simulink model "RobustFormationControl_FractionalModel_under_Dis"  (R2023a)
settings: Solver=ode3  StartTime=0.0  StopTime=30  FixedStep=0.0001  RelTol=1e-3
InitFcn:
  | % close all;
  | % clear all;
  | % clc;
  | % System & Qaudrotor Parameters
  | %==============================
  | m = 0.486;                                         % Quadrotor Mass ( kg )
  | 
  | L = 0.25;                                         % Length of the arm ( m )
  | % L = 0.25;                                         % Length of the arm ( m )
  | 
  | Ixx = 4.856e-03; Iyy = 4.856e-03; Izz = 8.801e-03; % The moments of inertia around x,y and z axes respectively ( kg.m^2 )
  | % Ixx = 3.8278e-03; Iyy = 3.8278e-03; Izz = 7.6566e-03; % The moments of inertia around x,y and z axes respectively ( kg.m^2 )
  | 
  | Jr = 2.8385e-5;                                            % The inertia moment of rotor ( kg.m^2 )
  | % Jr = 0;
  | 
  | % Kx=5.5670e-4;
  | % Ky=5.5670e-4;
  | % Kz=6.3540e-4;
  | % kx=0.032;
  | % ky=0.032;
  | % kz=0.048;
  | Kfx = 5.5670e-4; Kfy = 5.5670e-4; Kfz = 6.3540e-4;% The Rotational drag cofficients ( N/rad/s )
  | 
  | % Ktx = 0.032; Kty = 0.032; Ktz = 0.048;               % The linear drag coefficients in x, y, z respectively ( N/m/s )
  | Ktx = 5.5670e-4; Kty =5.5670e-4; Ktz = 6.3540e-4;               % The linear drag coefficients in x, y, z respectively ( N/m/s )
  | 
  | b = 2.923e-05;                                      % The lift coefficient
  | % b = 2.9842e-05;                                      % The lift coefficient
  | 
  | d = 1.12e-06;                                       % The drag coefficient
  | % d = 3.2320e-07;                                       % The drag coefficient
  | 
  | g = 9.81;                                          % The acceleration due to gravity ( m/s^2 )
  | 
  | %-------- The Coefficients of Non-linear Equations of Quadrotor ( Page 11) -------
  | %--------------------------------------------------------------------------------
  | % Rotational Equations
  | %=====================
  | % Coefficients in ( eq1 ) >>..
  | a1 = (Iyy - Izz)/Ixx;
  | b1 = - Jr/Ixx;
  | c1 = - Kfx/Ixx;
  | d1 = L/Ixx;
  | 
  | % Coefficients in ( eq2 ) >>..
  | a2 = (Izz - Ixx)/Iyy;
  | b2 = Jr/Iyy;
  | c2 = - Kfy/Iyy;
  | d2 = L/Iyy;
  | 
  | % Coefficients in ( eq3 ) >>..
  | a3 = (Ixx - Iyy)/Izz;
  | b3 = - Kfz/Izz;
  | c3 = 1/Izz;
  | % c3 = d/Izz;
  | 
  | % Translational Equations
  | %========================
  | % Coefficients in ( eq4 ) >>..
  | a4 = - Ktx/m;
  | % a4 =0;
  | % b4 = L/m;
  | b4 = 1/m;
  | 
  | % Coefficients in ( eq5 ) >>..
  | a5 = - Kty/m;
  | b5 = 1/m;
  | % b5 = L/m;
  | 
  | % Coefficients in ( eq6 ) >>..
  | a6 = - Ktz/m;
  | % a6 = 0;
  | b6 = 1/m;
  | % b6 = L/m;
  | %=================
  | %=================
  | % Sliding Surfaces Parameters of Integer  Model - Rotational System >>...
  | % 10, 1
  | % 10, 0.1
  | k1 = 10; k2 = 0.01; % for S2 ( Roll Angle Sliding Surface  Param.) (200 , 0.5)
  | k3 = 10; k4 = 0.01; % for S4 ( Pitch Angle Sliding Surface  Param.)
  | k5 = 10; k6 = 0.01; % for S6 ( Yaw Angle Sliding Surface  Param.)
  | %--------------
  | 
  | % Sliding Modse Controller Parameters of Integer Model>>...
  | % 0.1 ; 20
  | % 100; 0.05
  | qPhi = 10; kPhi =150;  % for U2 (100,1)
  | qTheta = 10; kTheta = 150;  % for U3
  | qPsi = 10; kPsi = 150;  % for U4
  | %-----------------
  | %==========================================================================
  | %==========================================================================
  | % Sliding Surfaces Parameters of Fractional Model >>...
  | 
  | % S2, S4 and S6 have the same parameters of Sliding Surfaces with Integer Model
  | %--------------
  | % n = 0.1, nn = 0.1
  | % n = 0.5, nn = 10;
  | % n = 0.25, nn = 15;
  | 
  | % n = 0.3;
  | % nn = 21.3;
  | % (0.5, 50)
  | n = 0.01;
  | nn = 3;
  | % for S8 ( x Position Sliding Surfece  Param.) (500, 1)
  | % 10, 0.1
  | q7 = 1*nn; q8 = 1*n; q9 = 1*n; q10 = 1*n;
  | % for S10 ( y Position Sliding Surfece  Param.) (500, 1)
  | q11 = 1*nn; q12 = 1*n; q13 = 1*n; q14 = 1*n;
  | % for S12 ( z Position Sliding Surfece  Param.) (500, 1)
  | q15 = 1*nn; q16 = 1*n; q17 = 1*n; q18 = 1*n;
  | %-------------------------------------------------------------------------
  | % Sliding Mode Controller Parameters of Fractional Model>>...
  | % 0.1, 10
  | % 1, 15
  | % ( 10, 20)
  | gX = 1; sX = 200; % for Ux (10,100)
  | gY = 1; sY = 200; % for Uy (10,100)
  | gZ = 1; sZ = 200; % for U1 (10,100)
  | %-------------------------------------------------------------------------
  | %-------------------------------------------------------------------------
  | %-------------------------------------------------------------------------
  | %-------------------------------------------------------------------------
  | %-------------------------------------------------------------------------
  | %-------------------------------------------------------------------------
  | % Control Design Parameters for the followers:
  | %==============================================
  | % % Parameters for the fractional order NTFSMC:
  | % Sliding Surface " Sx, Sy, and Sz ":
  | %------------------------
  | cx = 50*[4 4 4];
  | cxx = 0.01*[0.01 0.01 0.01];
  | 
  | cx1 = cx(1);
  | cy1 = cx(2);
  | cz1 = cx(3);
  | 
  | cx2 = cxx(1);
  | cy2 = cxx(2);
  | cz2 = cxx(3);
  | 
  | alpha1 = [0.7 0.7 0.7];
  | alpha2 = [0.01 0.01 0.01];
  | 
  | gammaX = [4 4 4];
  | gx  = gammaX(1);
  | gy = gammaX(2);
  | gz = gammaX(3);
  | 
  | p = 10;
  | q = 10;
  | 
  | % Sliding Surface " S_Phi , S_Theta, and  S_Psi":
  | %------------------------
  | cP = 50*[4 4 4];
  | cPP = 0.10*[0.01 0.01 0.01 0.01];
  | 
  | cPhi1 = cP(1);
  | cTheta1 = cP(2);
  | cPsi1 = cP(3);
  | 
  | cPhi2 = cPP(1);
  | cTheta2 = cPP(2);
  | cPsi2 = cPP(3);
  | gammaP = [4 4 4];
  | 
  | %=========================
  | %=========================
  | SigmaX = 1*[0.01 0.01 0.01];
  | SigmaXX = 0.1*[1 1 1];
  | 
  | Sigma1X = SigmaX(1);
  | Sigma1Y = SigmaX(2);
  | Sigma1Z = SigmaX(3);
  | %-----
  | Sigma2X = SigmaXX(1);
  | Sigma2Y = SigmaXX(2);
  | Sigma2Z = SigmaXX(3);
  | 
  | 
  | SigmaP = 0.01*[0.01 0.01 0.01];
  | SigmaPP =100*[1 1 1];
  | 
  | Sigma1Phi   = SigmaP(1);
  | Sigma1Theta = SigmaP(2);
  | Sigma1Psi   = SigmaP(3);
  | %----
  | Sigma2Phi   = SigmaPP(1);
  | Sigma2Theta = SigmaPP(2);
  | Sigma2Psi   = SigmaPP(3);
  | 
  | q0 = 0.01;
  | q1 = 0.01;
  | q2 = 0.01;
  | w = 0;
  | %=========================================
  | %=========================================
  | %=========================================
  | %=========================================
  | %=========================================
  | %=========================================
  | %=========================================
  | %=========================================
  | % The value of Beta ( The fractional order of the FOSMCs)
  | Beta = 0.2;
  | % The value of Disturbance:
  | Dis = 1;
  | dis = 0;
libraries: fod x135, eeStairGenerator x5
(part 1 of 10)
settings Model: Creator=jofan  LastModifiedBy=jofan
settings DataIOCC: ReturnWorkspaceOutputs=off

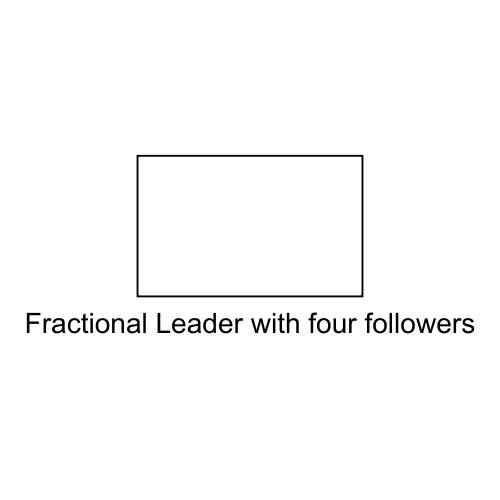
[thumbnail: Simulink's stored preview of the top-level diagram]
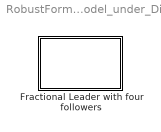
== system RobustFormationControl_FractionalModel_under_Dis ==
  Fractional Leader with four followers : Subsystem

== system RobustFormationControl_FractionalModel_under_Dis/Fractional Leader with four followers ==
  Follower 1 System : Subsystem
  Follower 2 System : Subsystem
  Follower 3 System : Subsystem
  Follower 4 System : Subsystem
  Fractional Model of the Leader : Subsystem
  Mux{,1..3} (4 alike) : Mux  Inputs=3
  dX : Constant  Value=-2
  dX1 : Constant  Value=-2
  dX2 : Constant  Value=-4
  dX3 : Constant  Value=-4
  dY : Constant  Value=2
  dY1 : Constant  Value=-2
  dY2 : Constant  Value=4
  dY3 : Constant  Value=-4
  dZ{,1..3} (4 alike) : Constant  Value=0
  wires:
  dY/1 -> Mux/2
  dZ/1 -> Mux/3
  dX/1 -> Mux/1
  dY1/1 -> Mux1/2
  dZ1/1 -> Mux1/3
  dX1/1 -> Mux1/1
  dX2/1 -> Mux2/1
  dZ2/1 -> Mux2/3
  dY2/1 -> Mux2/2
  dY3/1 -> Mux3/2
  dZ3/1 -> Mux3/3
  dX3/1 -> Mux3/1
  Mux/1 -> [dXYZ]
  Mux1/1 -> [dXYZ1]
  Mux2/1 -> [dXYZ2]
  Mux3/1 -> [dXYZ3]
  Fractional Model of the Leader/1(xLeader) -> [xyzL]
  [xyzL] -> Follower 1 System/1(xLeader)
  [xyzL] -> Follower 2 System/1(xLeader)
  [xyzL] -> Follower 4 System/1(xLeader)
  [xyzL] -> Follower 3 System/1(xLeader)
  [dXYZ] -> Follower 1 System/2(dXYZ)
  [dXYZ2] -> Follower 3 System/2(dXYZ)
  [dXYZ1] -> Follower 2 System/2(dXYZ)
  [dXYZ3] -> Follower 4 System/2(dXYZ)

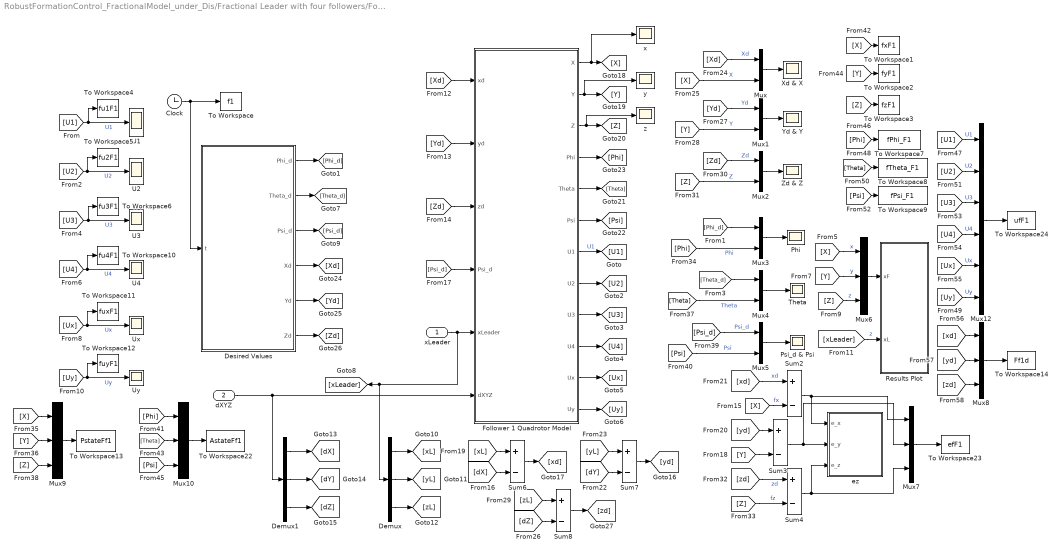
== system RobustFormationControl_FractionalModel_under_Dis/Fractional Leader with four followers/Follower 1 System ==
  xLeader : Inport
  dXYZ : Inport  Port=2
  " Phi " : Scope
  Clock : Clock
  Demux : Demux  Outputs=3
  Demux1 : Demux  Outputs=3
  Desired Values : Subsystem
  Follower 1 Quadrotor Model : Subsystem
  Mux{,1..5} (6 alike) : Mux  Inputs=2
  Mux{6..10} (5 alike) : Mux  Inputs=3
  Mux12 : Mux  Inputs=6
  Psi_d & Psi : Scope
  Results Plot : Subsystem
  Sum{2..4,6..8} (6 alike) : Sum  Inputs=+-
  "Theta " : Scope
  To Workspace : ToWorkspace  VariableName=f1  SampleTime=0.03
  To Workspace1 : ToWorkspace  VariableName=fxF1  SampleTime=0.03
  To Workspace10 : ToWorkspace  VariableName=fu4F1  SampleTime=0.03
  To Workspace11 : ToWorkspace  VariableName=fuxF1  SampleTime=0.03
  To Workspace12 : ToWorkspace  VariableName=fuyF1  SampleTime=0.03
  To Workspace13 : ToWorkspace  VariableName=PstateFf1  SampleTime=-1
  To Workspace14 : ToWorkspace  VariableName=Ff1d  SampleTime=-1
  To Workspace2 : ToWorkspace  VariableName=fyF1  SampleTime=0.03
  To Workspace22 : ToWorkspace  VariableName=AstateFf1  SampleTime=-1
  To Workspace23 : ToWorkspace  VariableName=efF1  SampleTime=-1
  To Workspace24 : ToWorkspace  VariableName=ufF1  SampleTime=-1
  To Workspace3 : ToWorkspace  VariableName=fzF1  SampleTime=0.03
  To Workspace4 : ToWorkspace  VariableName=fu1F1  SampleTime=0.03
  To Workspace5 : ToWorkspace  VariableName=fu2F1  SampleTime=0.03
  To Workspace6 : ToWorkspace  VariableName=fu3F1  SampleTime=0.03
  To Workspace7 : ToWorkspace  VariableName=fPhi_F1  SampleTime=0.03
  To Workspace8 : ToWorkspace  VariableName=fTheta_F1  SampleTime=0.03
  To Workspace9 : ToWorkspace  VariableName=fPsi_F1  SampleTime=0.03
  "U1 " : Scope
  U2 : Scope
  "U3 " : Scope
  "U4 " : Scope
  Ux : Scope
  Uy : Scope
  "Xd & X " : Scope
  Yd & Y : Scope
  "Zd & Z " : Scope
  ez : Subsystem
  x : Scope
  y : Scope
  z : Scope
  wires:
  Mux4/1 -> "Theta "/1
  [U2] -> To Workspace5/1, U2/1  "U2"
  [Yd] -> Mux1/1  "Yd"
  Follower 1 Quadrotor Model/10(U4) -> [U4]
  [Zd] -> Follower 1 Quadrotor Model/3(zd)
  [U4] -> To Workspace10/1, "U4 "/1  "U4"
  [Psi] -> To Workspace9/1
  [Z] -> Mux2/2  "Z"
  Follower 1 Quadrotor Model/2(Y) -> y/1, [Y]
  Clock/1 -> To Workspace/1, Desired Values/1(t)
  Follower 1 Quadrotor Model/7(U1) -> [U1]  "U1"
  Desired Values/2(Theta_d) -> [Theta_d]
  Mux2/1 -> "Zd & Z "/1
  [Theta] -> To Workspace8/1
  [Xd] -> Mux/1  "Xd"
  Follower 1 Quadrotor Model/12(Uy) -> [Uy]
  [Y] -> To Workspace2/1
  Follower 1 Quadrotor Model/11(Ux) -> [Ux]
  [X] -> To Workspace1/1
  [Yd] -> Follower 1 Quadrotor Model/2(yd)
  Mux/1 -> "Xd & X "/1
  Follower 1 Quadrotor Model/1(X) -> x/1, [X]
  Mux3/1 -> " Phi "/1
  Follower 1 Quadrotor Model/5(Theta) -> [Theta]
  Mux5/1 -> Psi_d & Psi/1
  [X] -> Mux/2  "X"
  Follower 1 Quadrotor Model/9(U3) -> [U3]
  [Theta] -> Mux4/2  "Theta"
  [Y] -> Mux1/2  "Y"
  [Uy] -> To Workspace12/1, Uy/1  "Uy"
  Desired Values/3(Psi_d) -> [Psi_d]
  Follower 1 Quadrotor Model/3(Z) -> z/1, [Z]
  [U1] -> To Workspace4/1, "U1 "/1  "U1"
  [Ux] -> To Workspace11/1, Ux/1  "Ux"
  Desired Values/6(Zd) -> [Zd]
  [Phi] -> Mux3/2  "Phi"
  Mux1/1 -> Yd & Y/1
  [Xd] -> Follower 1 Quadrotor Model/1(xd)
  [Psi] -> Mux5/2  "Psi"
  [Z] -> To Workspace3/1
  Follower 1 Quadrotor Model/8(U2) -> [U2]
  [Theta_d] -> Mux4/1
  [Psi_d] -> Mux5/1  "Psi_d"
  [Zd] -> Mux2/1  "Zd"
  [U3] -> To Workspace6/1, "U3 "/1  "U3"
  Desired Values/5(Yd) -> [Yd]
  [Psi_d] -> Follower 1 Quadrotor Model/4(Psi_d)
  Follower 1 Quadrotor Model/6(Psi) -> [Psi]
  Follower 1 Quadrotor Model/4(Phi) -> [Phi]
  Desired Values/4(Xd) -> [Xd]
  [Phi_d] -> Mux3/1
  Desired Values/1(Phi_d) -> [Phi_d]
  [Phi] -> To Workspace7/1
  xLeader/1 -> Demux/1, [xLeader], Follower 1 Quadrotor Model/5(xLeader)
  [Z] -> Mux6/3  "z"
  [X] -> Mux6/1  "x"
  [xLeader] -> Results Plot/2(xL)  "z"
  Mux6/1 -> Results Plot/1(xF)
  [Y] -> Mux6/2  "y"
  dXYZ/1 -> Demux1/1, Follower 1 Quadrotor Model/6(dXYZ)
  Demux/1 -> [xL]
  Demux/3 -> [zL]
  Demux/2 -> [yL]
  Demux1/3 -> [dZ]
  Demux1/2 -> [dY]
  Demux1/1 -> [dX]
  [xL] -> Sum6/1
  [dX] -> Sum6/2
  [dY] -> Sum7/2
  [yL] -> Sum7/1
  [dZ] -> Sum8/2
  [zL] -> Sum8/1
  Sum7/1 -> [yd]
  Sum6/1 -> [xd]
  Sum8/1 -> [zd]
  [yd] -> Mux8/2
  [zd] -> Sum4/1  "zd"
  [Z] -> Mux9/3
  [Uy] -> Mux12/6  "Uy"
  [Z] -> Sum4/2  "fz"
  [X] -> Mux9/1
  [U2] -> Mux12/2  "U2"
  [Ux] -> Mux12/5  "Ux"
  [U1] -> Mux12/1  "U1"
  [Y] -> Mux9/2
  Sum3/1 -> Mux7/2, ez/2(e_y)
  [Y] -> Sum3/2
  Sum2/1 -> Mux7/1, ez/1(e_x)
  Sum4/1 -> Mux7/3, ez/3(e_z)
  [yd] -> Sum3/1
  Mux12/1 -> To Workspace24/1
  [Theta] -> Mux10/2
  [Psi] -> Mux10/3
  Mux7/1 -> To Workspace23/1
  [zd] -> Mux8/3
  Mux8/1 -> To Workspace14/1
  [X] -> Sum2/2  "fx"
  Mux10/1 -> To Workspace22/1
  Mux9/1 -> To Workspace13/1
  [Phi] -> Mux10/1
  [U4] -> Mux12/4  "U4"
  [xd] -> Mux8/1
  [U3] -> Mux12/3  "U3"
  [xd] -> Sum2/1  "xd"

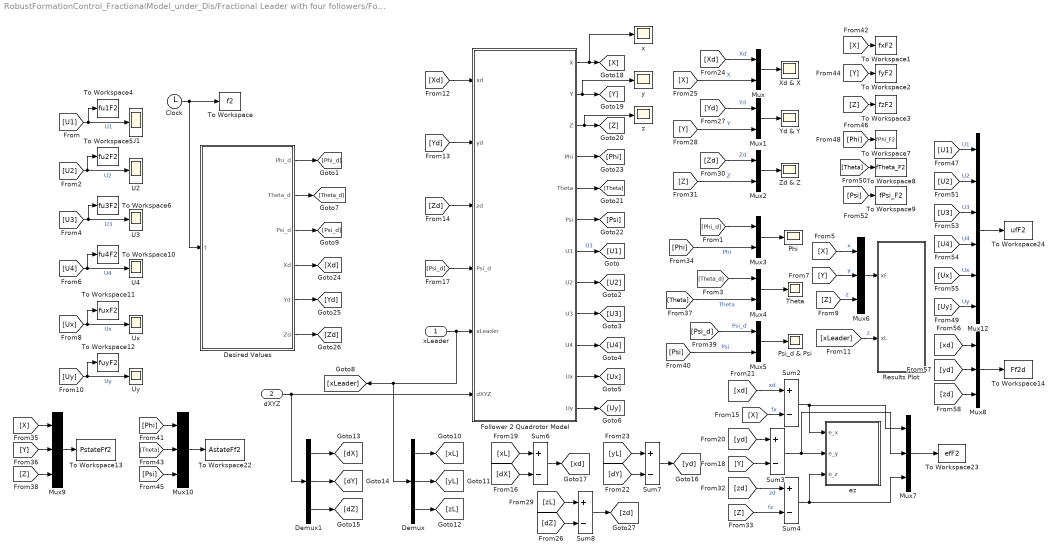
== system RobustFormationControl_FractionalModel_under_Dis/Fractional Leader with four followers/Follower 2 System ==
  xLeader : Inport
  dXYZ : Inport  Port=2
  " Phi " : Scope
  Clock : Clock
  Demux : Demux  Outputs=3
  Demux1 : Demux  Outputs=3
  Desired Values : Subsystem
  Follower 2 Quadrotor Model : Subsystem
  Mux{,1..5} (6 alike) : Mux  Inputs=2
  Mux{6..10} (5 alike) : Mux  Inputs=3
  Mux12 : Mux  Inputs=6
  Psi_d & Psi : Scope
  Results Plot : Subsystem
  Sum{2..4,6..8} (6 alike) : Sum  Inputs=+-
  "Theta " : Scope
  To Workspace : ToWorkspace  VariableName=f2  SampleTime=0.03
  To Workspace1 : ToWorkspace  VariableName=fxF2  SampleTime=0.03
  To Workspace10 : ToWorkspace  VariableName=fu4F2  SampleTime=0.03
  To Workspace11 : ToWorkspace  VariableName=fuxF2  SampleTime=0.03
  To Workspace12 : ToWorkspace  VariableName=fuyF2  SampleTime=0.03
  To Workspace13 : ToWorkspace  VariableName=PstateFf2  SampleTime=-1
  To Workspace14 : ToWorkspace  VariableName=Ff2d  SampleTime=-1
  To Workspace2 : ToWorkspace  VariableName=fyF2  SampleTime=0.03
  To Workspace22 : ToWorkspace  VariableName=AstateFf2  SampleTime=-1
  To Workspace23 : ToWorkspace  VariableName=efF2  SampleTime=-1
  To Workspace24 : ToWorkspace  VariableName=ufF2  SampleTime=-1
  To Workspace3 : ToWorkspace  VariableName=fzF2  SampleTime=0.03
  To Workspace4 : ToWorkspace  VariableName=fu1F2  SampleTime=0.03
  To Workspace5 : ToWorkspace  VariableName=fu2F2  SampleTime=0.03
  To Workspace6 : ToWorkspace  VariableName=fu3F2  SampleTime=0.03
  To Workspace7 : ToWorkspace  VariableName=fPhi_F2  SampleTime=0.03
  To Workspace8 : ToWorkspace  VariableName=fTheta_F2  SampleTime=0.03
  To Workspace9 : ToWorkspace  VariableName=fPsi_F2  SampleTime=0.03
  "U1 " : Scope
  U2 : Scope
  "U3 " : Scope
  "U4 " : Scope
  Ux : Scope
  Uy : Scope
  "Xd & X " : Scope
  Yd & Y : Scope
  "Zd & Z " : Scope
  ez : Subsystem
  x : Scope
  y : Scope
  z : Scope
  wires:
  Mux4/1 -> "Theta "/1
  [U2] -> To Workspace5/1, U2/1  "U2"
  [Yd] -> Mux1/1  "Yd"
  Follower 2 Quadrotor Model/10(U4) -> [U4]
  [Zd] -> Follower 2 Quadrotor Model/3(zd)
  [U4] -> To Workspace10/1, "U4 "/1  "U4"
  [Psi] -> To Workspace9/1
  [Z] -> Mux2/2  "Z"
  Follower 2 Quadrotor Model/2(Y) -> y/1, [Y]
  Clock/1 -> To Workspace/1, Desired Values/1(t)
  Follower 2 Quadrotor Model/7(U1) -> [U1]  "U1"
  Desired Values/2(Theta_d) -> [Theta_d]
  Mux2/1 -> "Zd & Z "/1
  [Theta] -> To Workspace8/1
  [Xd] -> Mux/1  "Xd"
  Follower 2 Quadrotor Model/12(Uy) -> [Uy]
  [Y] -> To Workspace2/1
  Follower 2 Quadrotor Model/11(Ux) -> [Ux]
  [X] -> To Workspace1/1
  [Yd] -> Follower 2 Quadrotor Model/2(yd)
  Mux/1 -> "Xd & X "/1
  Follower 2 Quadrotor Model/1(X) -> x/1, [X]
  Mux3/1 -> " Phi "/1
  Follower 2 Quadrotor Model/5(Theta) -> [Theta]
  Mux5/1 -> Psi_d & Psi/1
  [X] -> Mux/2  "X"
  Follower 2 Quadrotor Model/9(U3) -> [U3]
  [Theta] -> Mux4/2  "Theta"
  [Y] -> Mux1/2  "Y"
  [Uy] -> To Workspace12/1, Uy/1  "Uy"
  Desired Values/3(Psi_d) -> [Psi_d]
  Follower 2 Quadrotor Model/3(Z) -> z/1, [Z]
  [U1] -> To Workspace4/1, "U1 "/1  "U1"
  [Ux] -> To Workspace11/1, Ux/1  "Ux"
  Desired Values/6(Zd) -> [Zd]
  [Phi] -> Mux3/2  "Phi"
  Mux1/1 -> Yd & Y/1
  [Xd] -> Follower 2 Quadrotor Model/1(xd)
  [Psi] -> Mux5/2  "Psi"
  [Z] -> To Workspace3/1
  Follower 2 Quadrotor Model/8(U2) -> [U2]
  [Theta_d] -> Mux4/1
  [Psi_d] -> Mux5/1  "Psi_d"
  [Zd] -> Mux2/1  "Zd"
  [U3] -> To Workspace6/1, "U3 "/1  "U3"
  Desired Values/5(Yd) -> [Yd]
  [Psi_d] -> Follower 2 Quadrotor Model/4(Psi_d)
  Follower 2 Quadrotor Model/6(Psi) -> [Psi]
  Follower 2 Quadrotor Model/4(Phi) -> [Phi]
  Desired Values/4(Xd) -> [Xd]
  [Phi_d] -> Mux3/1
  Desired Values/1(Phi_d) -> [Phi_d]
  [Phi] -> To Workspace7/1
  [Z] -> Mux6/3  "z"
  [X] -> Mux6/1  "x"
  [xLeader] -> Results Plot/2(xL)  "z"
  Mux6/1 -> Results Plot/1(xF)
  [Y] -> Mux6/2  "y"
  Demux1/3 -> [dZ]
  Demux/2 -> [yL]
  Sum8/1 -> [zd]
  [dZ] -> Sum8/2
  [dX] -> Sum6/2
  dXYZ/1 -> Demux1/1, Follower 2 Quadrotor Model/6(dXYZ)
  [zL] -> Sum8/1
  Sum7/1 -> [yd]
  [yL] -> Sum7/1
  Demux/3 -> [zL]
  [dY] -> Sum7/2
  Demux1/1 -> [dX]
  Demux/1 -> [xL]
  Sum6/1 -> [xd]
  xLeader/1 -> [xLeader], Demux/1, Follower 2 Quadrotor Model/5(xLeader)
  Demux1/2 -> [dY]
  [xL] -> Sum6/1
  [Z] -> Mux9/3
  [zd] -> Sum4/1  "zd"
  [Phi] -> Mux10/1
  [U3] -> Mux12/3  "U3"
  [xd] -> Mux8/1
  Mux9/1 -> To Workspace13/1
  [Theta] -> Mux10/2
  Mux7/1 -> To Workspace23/1
  [X] -> Sum2/2  "fx"
  [Psi] -> Mux10/3
  Mux8/1 -> To Workspace14/1
  Sum2/1 -> Mux7/1, ez/1(e_x)
  [U4] -> Mux12/4  "U4"
  Sum4/1 -> Mux7/3, ez/3(e_z)
  Mux12/1 -> To Workspace24/1
  Sum3/1 -> Mux7/2, ez/2(e_y)
  [Y] -> Sum3/2
  Mux10/1 -> To Workspace22/1
  [U2] -> Mux12/2  "U2"
  [zd] -> Mux8/3
  [Y] -> Mux9/2
  [Ux] -> Mux12/5  "Ux"
  [yd] -> Mux8/2
  [X] -> Mux9/1
  [Uy] -> Mux12/6  "Uy"
  [yd] -> Sum3/1
  [U1] -> Mux12/1  "U1"
  [Z] -> Sum4/2  "fz"
  [xd] -> Sum2/1  "xd"

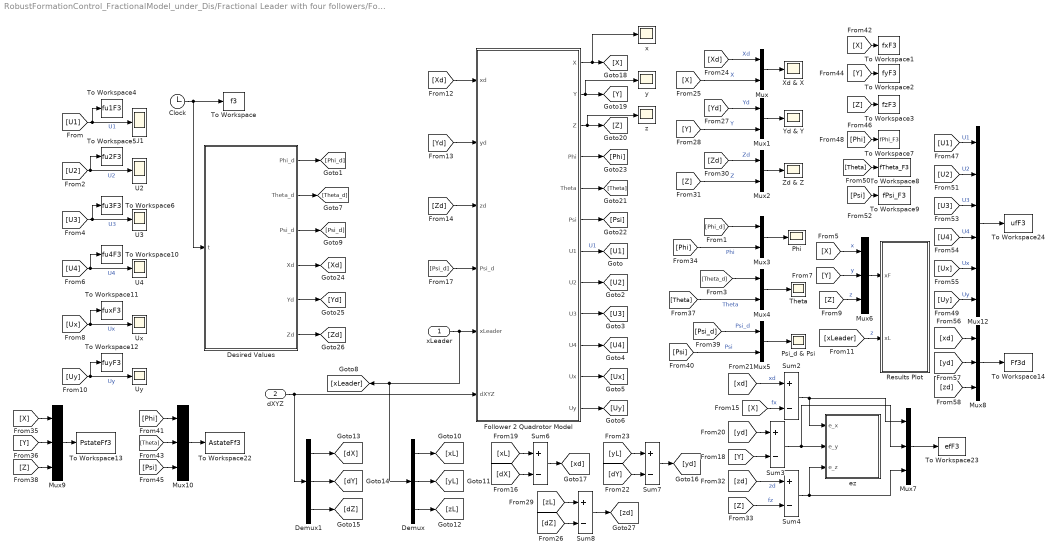
== system RobustFormationControl_FractionalModel_under_Dis/Fractional Leader with four followers/Follower 3 System ==
  xLeader : Inport
  dXYZ : Inport  Port=2
  " Phi " : Scope
  Clock : Clock
  Demux : Demux  Outputs=3
  Demux1 : Demux  Outputs=3
  Desired Values : Subsystem
  Follower 2 Quadrotor Model : Subsystem
  Mux{,1..5} (6 alike) : Mux  Inputs=2
  Mux{6..10} (5 alike) : Mux  Inputs=3
  Mux12 : Mux  Inputs=6
  Psi_d & Psi : Scope
  Results Plot : Subsystem
  Sum{2..4,6..8} (6 alike) : Sum  Inputs=+-
  "Theta " : Scope
  To Workspace : ToWorkspace  VariableName=f3  SampleTime=0.03
  To Workspace1 : ToWorkspace  VariableName=fxF3  SampleTime=0.03
  To Workspace10 : ToWorkspace  VariableName=fu4F3  SampleTime=0.03
  To Workspace11 : ToWorkspace  VariableName=fuxF3  SampleTime=0.03
  To Workspace12 : ToWorkspace  VariableName=fuyF3  SampleTime=0.03
  To Workspace13 : ToWorkspace  VariableName=PstateFf3  SampleTime=-1
  To Workspace14 : ToWorkspace  VariableName=Ff3d  SampleTime=-1
  To Workspace2 : ToWorkspace  VariableName=fyF3  SampleTime=0.03
  To Workspace22 : ToWorkspace  VariableName=AstateFf3  SampleTime=-1
  To Workspace23 : ToWorkspace  VariableName=efF3  SampleTime=-1
  To Workspace24 : ToWorkspace  VariableName=ufF3  SampleTime=-1
  To Workspace3 : ToWorkspace  VariableName=fzF3  SampleTime=0.03
  To Workspace4 : ToWorkspace  VariableName=fu1F3  SampleTime=0.03
  To Workspace5 : ToWorkspace  VariableName=fu2F3  SampleTime=0.03
  To Workspace6 : ToWorkspace  VariableName=fu3F3  SampleTime=0.03
  To Workspace7 : ToWorkspace  VariableName=fPhi_F3  SampleTime=0.03
  To Workspace8 : ToWorkspace  VariableName=fTheta_F3  SampleTime=0.03
  To Workspace9 : ToWorkspace  VariableName=fPsi_F3  SampleTime=0.03
  "U1 " : Scope
  U2 : Scope
  "U3 " : Scope
  "U4 " : Scope
  Ux : Scope
  Uy : Scope
  "Xd & X " : Scope
  Yd & Y : Scope
  "Zd & Z " : Scope
  ez : Subsystem
  x : Scope
  y : Scope
  z : Scope
  wires:
  [Y] -> Mux6/2  "y"
  Mux6/1 -> Results Plot/1(xF)
  [xLeader] -> Results Plot/2(xL)  "z"
  [X] -> Mux6/1  "x"
  [Z] -> Mux6/3  "z"
  xLeader/1 -> Follower 2 Quadrotor Model/5(xLeader), Demux/1, [xLeader]
  [Phi] -> To Workspace7/1
  Desired Values/1(Phi_d) -> [Phi_d]
  [Phi_d] -> Mux3/1
  Desired Values/4(Xd) -> [Xd]
  Follower 2 Quadrotor Model/4(Phi) -> [Phi]
  Follower 2 Quadrotor Model/6(Psi) -> [Psi]
  [Psi_d] -> Follower 2 Quadrotor Model/4(Psi_d)
  Desired Values/5(Yd) -> [Yd]
  [U3] -> "U3 "/1, To Workspace6/1  "U3"
  [Zd] -> Mux2/1  "Zd"
  [Psi_d] -> Mux5/1  "Psi_d"
  [Theta_d] -> Mux4/1
  Follower 2 Quadrotor Model/8(U2) -> [U2]
  [Z] -> To Workspace3/1
  [Psi] -> Mux5/2  "Psi"
  [Xd] -> Follower 2 Quadrotor Model/1(xd)
  Mux1/1 -> Yd & Y/1
  [Phi] -> Mux3/2  "Phi"
  Desired Values/6(Zd) -> [Zd]
  [Ux] -> Ux/1, To Workspace11/1  "Ux"
  [U1] -> "U1 "/1, To Workspace4/1  "U1"
  Follower 2 Quadrotor Model/3(Z) -> [Z], z/1
  Desired Values/3(Psi_d) -> [Psi_d]
  [Uy] -> Uy/1, To Workspace12/1  "Uy"
  [Y] -> Mux1/2  "Y"
  [Theta] -> Mux4/2  "Theta"
  Follower 2 Quadrotor Model/9(U3) -> [U3]
  [X] -> Mux/2  "X"
  Mux5/1 -> Psi_d & Psi/1
  Follower 2 Quadrotor Model/5(Theta) -> [Theta]
  Mux3/1 -> " Phi "/1
  Follower 2 Quadrotor Model/1(X) -> [X], x/1
  Mux/1 -> "Xd & X "/1
  [Yd] -> Follower 2 Quadrotor Model/2(yd)
  [X] -> To Workspace1/1
  Follower 2 Quadrotor Model/11(Ux) -> [Ux]
  [Y] -> To Workspace2/1
  Follower 2 Quadrotor Model/12(Uy) -> [Uy]
  [Xd] -> Mux/1  "Xd"
  [Theta] -> To Workspace8/1
  Mux2/1 -> "Zd & Z "/1
  Desired Values/2(Theta_d) -> [Theta_d]
  Follower 2 Quadrotor Model/7(U1) -> [U1]  "U1"
  Clock/1 -> Desired Values/1(t), To Workspace/1
  Follower 2 Quadrotor Model/2(Y) -> [Y], y/1
  [Z] -> Mux2/2  "Z"
  [Psi] -> To Workspace9/1
  [U4] -> "U4 "/1, To Workspace10/1  "U4"
  [Zd] -> Follower 2 Quadrotor Model/3(zd)
  Follower 2 Quadrotor Model/10(U4) -> [U4]
  [Yd] -> Mux1/1  "Yd"
  [U2] -> U2/1, To Workspace5/1  "U2"
  Mux4/1 -> "Theta "/1
  Demux1/3 -> [dZ]
  Demux/2 -> [yL]
  Sum8/1 -> [zd]
  [dZ] -> Sum8/2
  [dX] -> Sum6/2
  dXYZ/1 -> Demux1/1, Follower 2 Quadrotor Model/6(dXYZ)
  [zL] -> Sum8/1
  Sum7/1 -> [yd]
  [yL] -> Sum7/1
  Demux/3 -> [zL]
  [dY] -> Sum7/2
  Demux1/1 -> [dX]
  Demux/1 -> [xL]
  Sum6/1 -> [xd]
  Demux1/2 -> [dY]
  [xL] -> Sum6/1
  [Z] -> Mux9/3
  [zd] -> Sum4/1  "zd"
  [Phi] -> Mux10/1
  [U3] -> Mux12/3  "U3"
  [xd] -> Mux8/1
  Mux9/1 -> To Workspace13/1
  [Theta] -> Mux10/2
  Mux7/1 -> To Workspace23/1
  [X] -> Sum2/2  "fx"
  [Psi] -> Mux10/3
  Mux8/1 -> To Workspace14/1
  Sum2/1 -> Mux7/1, ez/1(e_x)
  [U4] -> Mux12/4  "U4"
  Sum4/1 -> Mux7/3, ez/3(e_z)
  Mux12/1 -> To Workspace24/1
  Sum3/1 -> Mux7/2, ez/2(e_y)
  [Y] -> Sum3/2
  Mux10/1 -> To Workspace22/1
  [U2] -> Mux12/2  "U2"
  [zd] -> Mux8/3
  [Y] -> Mux9/2
  [Ux] -> Mux12/5  "Ux"
  [yd] -> Mux8/2
  [X] -> Mux9/1
  [Uy] -> Mux12/6  "Uy"
  [yd] -> Sum3/1
  [U1] -> Mux12/1  "U1"
  [Z] -> Sum4/2  "fz"
  [xd] -> Sum2/1  "xd"

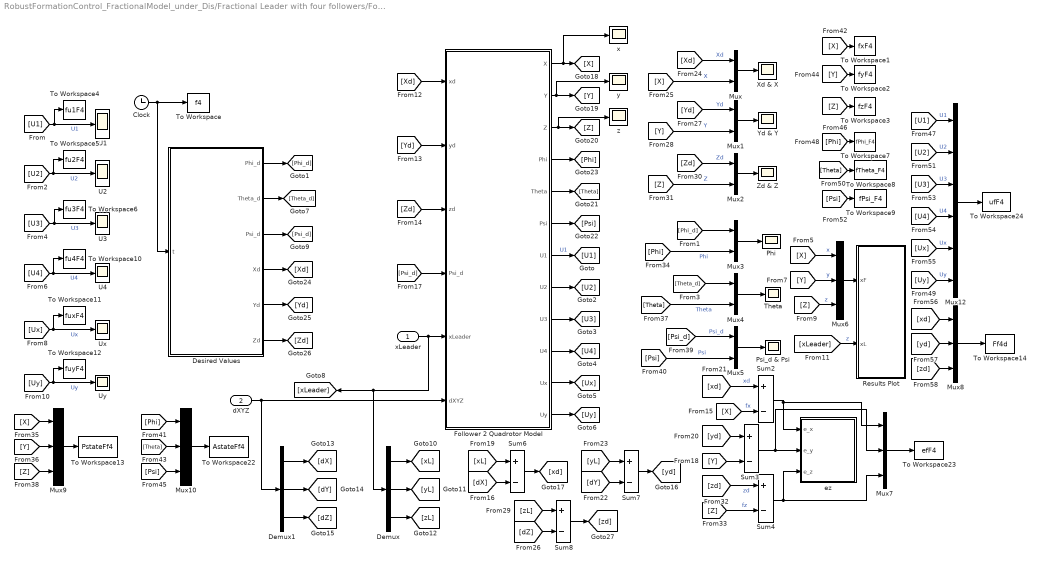
== system RobustFormationControl_FractionalModel_under_Dis/Fractional Leader with four followers/Follower 4 System ==
  xLeader : Inport
  dXYZ : Inport  Port=2
  " Phi " : Scope
  Clock : Clock
  Demux : Demux  Outputs=3
  Demux1 : Demux  Outputs=3
  Desired Values : Subsystem
  Follower 2 Quadrotor Model : Subsystem
  Mux{,1..5} (6 alike) : Mux  Inputs=2
  Mux{6..10} (5 alike) : Mux  Inputs=3
  Mux12 : Mux  Inputs=6
  Psi_d & Psi : Scope
  Results Plot : Subsystem
  Sum{2..4,6..8} (6 alike) : Sum  Inputs=+-
  "Theta " : Scope
  To Workspace : ToWorkspace  VariableName=f4  SampleTime=0.03
  To Workspace1 : ToWorkspace  VariableName=fxF4  SampleTime=0.03
  To Workspace10 : ToWorkspace  VariableName=fu4F4  SampleTime=0.03
  To Workspace11 : ToWorkspace  VariableName=fuxF4  SampleTime=0.03
  To Workspace12 : ToWorkspace  VariableName=fuyF4  SampleTime=0.03
  To Workspace13 : ToWorkspace  VariableName=PstateFf4  SampleTime=-1
  To Workspace14 : ToWorkspace  VariableName=Ff4d  SampleTime=-1
  To Workspace2 : ToWorkspace  VariableName=fyF4  SampleTime=0.03
  To Workspace22 : ToWorkspace  VariableName=AstateFf4  SampleTime=-1
  To Workspace23 : ToWorkspace  VariableName=efF4  SampleTime=-1
  To Workspace24 : ToWorkspace  VariableName=ufF4  SampleTime=-1
  To Workspace3 : ToWorkspace  VariableName=fzF4  SampleTime=0.03
  To Workspace4 : ToWorkspace  VariableName=fu1F4  SampleTime=0.03
  To Workspace5 : ToWorkspace  VariableName=fu2F4  SampleTime=0.03
  To Workspace6 : ToWorkspace  VariableName=fu3F4  SampleTime=0.03
  To Workspace7 : ToWorkspace  VariableName=fPhi_F4  SampleTime=0.03
  To Workspace8 : ToWorkspace  VariableName=fTheta_F4  SampleTime=0.03
  To Workspace9 : ToWorkspace  VariableName=fPsi_F4  SampleTime=0.03
  "U1 " : Scope
  U2 : Scope
  "U3 " : Scope
  "U4 " : Scope
  Ux : Scope
  Uy : Scope
  "Xd & X " : Scope
  Yd & Y : Scope
  "Zd & Z " : Scope
  ez : Subsystem
  x : Scope
  y : Scope
  z : Scope
  wires:
  Mux4/1 -> "Theta "/1
  [U2] -> To Workspace5/1, U2/1  "U2"
  [Yd] -> Mux1/1  "Yd"
  Follower 2 Quadrotor Model/10(U4) -> [U4]
  [Zd] -> Follower 2 Quadrotor Model/3(zd)
  [U4] -> To Workspace10/1, "U4 "/1  "U4"
  [Psi] -> To Workspace9/1
  [Z] -> Mux2/2  "Z"
  Follower 2 Quadrotor Model/2(Y) -> y/1, [Y]
  Clock/1 -> To Workspace/1, Desired Values/1(t)
  Follower 2 Quadrotor Model/7(U1) -> [U1]  "U1"
  Desired Values/2(Theta_d) -> [Theta_d]
  Mux2/1 -> "Zd & Z "/1
  [Theta] -> To Workspace8/1
  [Xd] -> Mux/1  "Xd"
  Follower 2 Quadrotor Model/12(Uy) -> [Uy]
  [Y] -> To Workspace2/1
  Follower 2 Quadrotor Model/11(Ux) -> [Ux]
  [X] -> To Workspace1/1
  [Yd] -> Follower 2 Quadrotor Model/2(yd)
  Mux/1 -> "Xd & X "/1
  Follower 2 Quadrotor Model/1(X) -> x/1, [X]
  Mux3/1 -> " Phi "/1
  Follower 2 Quadrotor Model/5(Theta) -> [Theta]
  Mux5/1 -> Psi_d & Psi/1
  [X] -> Mux/2  "X"
  Follower 2 Quadrotor Model/9(U3) -> [U3]
  [Theta] -> Mux4/2  "Theta"
  [Y] -> Mux1/2  "Y"
  [Uy] -> To Workspace12/1, Uy/1  "Uy"
  Desired Values/3(Psi_d) -> [Psi_d]
  Follower 2 Quadrotor Model/3(Z) -> z/1, [Z]
  [U1] -> To Workspace4/1, "U1 "/1  "U1"
  [Ux] -> To Workspace11/1, Ux/1  "Ux"
  Desired Values/6(Zd) -> [Zd]
  [Phi] -> Mux3/2  "Phi"
  Mux1/1 -> Yd & Y/1
  [Xd] -> Follower 2 Quadrotor Model/1(xd)
  [Psi] -> Mux5/2  "Psi"
  [Z] -> To Workspace3/1
  Follower 2 Quadrotor Model/8(U2) -> [U2]
  [Theta_d] -> Mux4/1
  [Psi_d] -> Mux5/1  "Psi_d"
  [Zd] -> Mux2/1  "Zd"
  [U3] -> To Workspace6/1, "U3 "/1  "U3"
  Desired Values/5(Yd) -> [Yd]
  [Psi_d] -> Follower 2 Quadrotor Model/4(Psi_d)
  Follower 2 Quadrotor Model/6(Psi) -> [Psi]
  Follower 2 Quadrotor Model/4(Phi) -> [Phi]
  Desired Values/4(Xd) -> [Xd]
  [Phi_d] -> Mux3/1
  Desired Values/1(Phi_d) -> [Phi_d]
  [Phi] -> To Workspace7/1
  xLeader/1 -> Demux/1, [xLeader], Follower 2 Quadrotor Model/5(xLeader)
  [Z] -> Mux6/3  "z"
  [X] -> Mux6/1  "x"
  [xLeader] -> Results Plot/2(xL)  "z"
  Mux6/1 -> Results Plot/1(xF)
  [Y] -> Mux6/2  "y"
  Demux1/3 -> [dZ]
  Demux/2 -> [yL]
  Sum8/1 -> [zd]
  [dZ] -> Sum8/2
  [dX] -> Sum6/2
  dXYZ/1 -> Demux1/1, Follower 2 Quadrotor Model/6(dXYZ)
  [zL] -> Sum8/1
  Sum7/1 -> [yd]
  [yL] -> Sum7/1
  Demux/3 -> [zL]
  [dY] -> Sum7/2
  Demux1/1 -> [dX]
  Demux/1 -> [xL]
  Sum6/1 -> [xd]
  Demux1/2 -> [dY]
  [xL] -> Sum6/1
  [Z] -> Mux9/3
  [zd] -> Sum4/1  "zd"
  [Phi] -> Mux10/1
  [U3] -> Mux12/3  "U3"
  [xd] -> Mux8/1
  Mux9/1 -> To Workspace13/1
  [Theta] -> Mux10/2
  Mux7/1 -> To Workspace23/1
  [X] -> Sum2/2  "fx"
  [Psi] -> Mux10/3
  Mux8/1 -> To Workspace14/1
  Sum2/1 -> Mux7/1, ez/1(e_x)
  [U4] -> Mux12/4  "U4"
  Sum4/1 -> Mux7/3, ez/3(e_z)
  Mux12/1 -> To Workspace24/1
  Sum3/1 -> Mux7/2, ez/2(e_y)
  [Y] -> Sum3/2
  Mux10/1 -> To Workspace22/1
  [U2] -> Mux12/2  "U2"
  [zd] -> Mux8/3
  [Y] -> Mux9/2
  [Ux] -> Mux12/5  "Ux"
  [yd] -> Mux8/2
  [X] -> Mux9/1
  [Uy] -> Mux12/6  "Uy"
  [yd] -> Sum3/1
  [U1] -> Mux12/1  "U1"
  [Z] -> Sum4/2  "fz"
  [xd] -> Sum2/1  "xd"

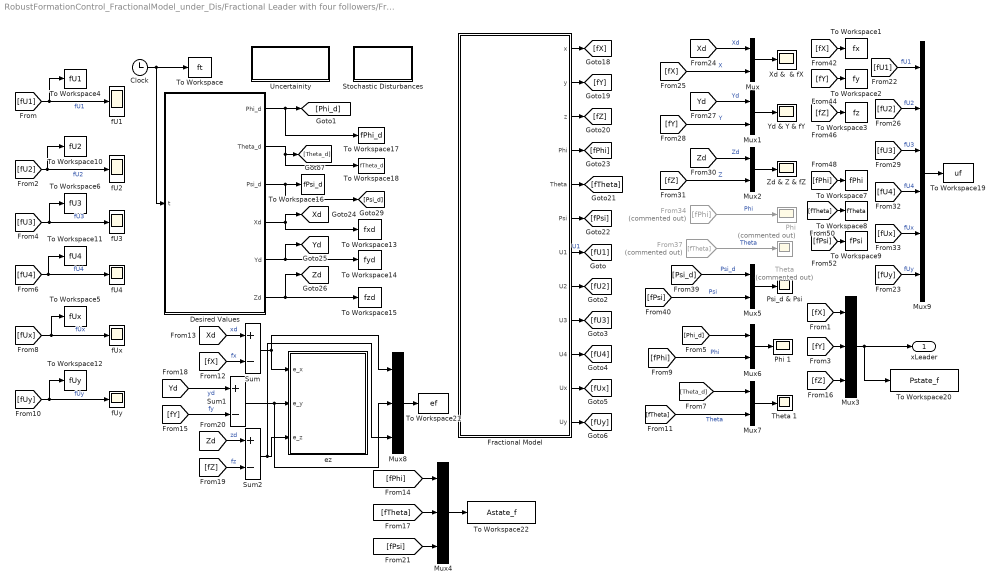
== system RobustFormationControl_FractionalModel_under_Dis/Fractional Leader with four followers/Fractional Model of the Leader ==
  " Phi " : Scope  Commented=on
  " Phi 1" : Scope
  Clock : Clock
  Desired Values : Subsystem
  Fractional Model : Subsystem
  From34 : From  Commented=on  GotoTag=fPhi
  From37 : From  Commented=on  GotoTag=fTheta
  Mux{,1..2,5..7} (6 alike) : Mux  Inputs=2
  Mux3 : Mux  Inputs=3
  Mux4 : Mux  Inputs=3
  Mux8 : Mux  Inputs=3
  Mux9 : Mux  Inputs=6
  Psi_d & Psi : Scope
  Stochastic Disturbances : Subsystem
  Sum : Sum  Inputs=+-
  Sum1 : Sum  Inputs=+-
  Sum2 : Sum  Inputs=+-
  "Theta " : Scope  Commented=on
  Theta 1 : Scope
  To Workspace : ToWorkspace  VariableName=ft  SampleTime=0.03
  To Workspace1 : ToWorkspace  VariableName=fx  SampleTime=0.03
  To Workspace10 : ToWorkspace  VariableName=fU2  SampleTime=0.03
  To Workspace11 : ToWorkspace  VariableName=fU4  SampleTime=0.03
  To Workspace12 : ToWorkspace  VariableName=fUy  SampleTime=0.03
  To Workspace13 : ToWorkspace  VariableName=fxd  SampleTime=0.03
  To Workspace14 : ToWorkspace  VariableName=fyd  SampleTime=0.03
  To Workspace15 : ToWorkspace  VariableName=fzd  SampleTime=0.03
  To Workspace16 : ToWorkspace  VariableName=fPsi_d  SampleTime=0.03
  To Workspace17 : ToWorkspace  VariableName=fPhi_d  SampleTime=0.03
  To Workspace18 : ToWorkspace  VariableName=fTheta_d  SampleTime=0.03
  To Workspace19 : ToWorkspace  VariableName=uf  SampleTime=-1
  To Workspace2 : ToWorkspace  VariableName=fy  SampleTime=0.03
  To Workspace20 : ToWorkspace  VariableName=Pstate_f  SampleTime=-1
  To Workspace21 : ToWorkspace  VariableName=ef  SampleTime=-1
  To Workspace22 : ToWorkspace  VariableName=Astate_f  SampleTime=-1
  To Workspace3 : ToWorkspace  VariableName=fz  SampleTime=0.03
  To Workspace4 : ToWorkspace  VariableName=fU1  SampleTime=0.03
  To Workspace5 : ToWorkspace  VariableName=fUx  SampleTime=0.03
  To Workspace6 : ToWorkspace  VariableName=fU3  SampleTime=0.03
  To Workspace7 : ToWorkspace  VariableName=fPhi  SampleTime=0.03
  To Workspace8 : ToWorkspace  VariableName=fTheta  SampleTime=0.03
  To Workspace9 : ToWorkspace  VariableName=fPsi  SampleTime=0.03
  Uncertainity : Subsystem
  Xd &  & fX : Scope
  Yd & Y & fY : Scope
  Zd & Z & fZ : Scope
  ez : Subsystem
  "fU1 " : Scope
  fU2 : Scope
  "fU3 " : Scope
  "fU4 " : Scope
  fUx : Scope
  fUy : Scope
  xLeader : Outport
  tag scope: Xd=global, Yd=global, Zd=global
  wires:
  Fractional Model/7(U1) -> [fU1]  "U1"
  [fU1] -> To Workspace4/1, "fU1 "/1  "fU1"
  Fractional Model/8(U2) -> [fU2]
  Fractional Model/9(U3) -> [fU3]
  Fractional Model/10(U4) -> [fU4]
  Fractional Model/11(Ux) -> [fUx]
  Fractional Model/12(Uy) -> [fUy]
  [fU2] -> To Workspace10/1, fU2/1  "fU2"
  [fU3] -> To Workspace6/1, "fU3 "/1  "fU3"
  [fU4] -> To Workspace11/1, "fU4 "/1  "fU4"
  [fUx] -> To Workspace5/1, fUx/1  "fUx"
  [fUy] -> To Workspace12/1, fUy/1  "fUy"
  Fractional Model/1(x) -> [fX]
  Fractional Model/2(y) -> [fY]
  Fractional Model/3(z) -> [fZ]
  Fractional Model/4(Phi) -> [fPhi]
  Fractional Model/5(Theta) -> [fTheta]
  Fractional Model/6(Psi) -> [fPsi]
  [fZ] -> Mux2/2  "Z"
  Mux2/1 -> Zd & Z & fZ/1
  [fX] -> Mux/2  "X"
  [Xd] -> Mux/1  "Xd"
  Mux/1 -> Xd &  & fX/1
  [Yd] -> Mux1/1  "Yd"
  Mux1/1 -> Yd & Y & fY/1
  [fY] -> Mux1/2  "Y"
  [Zd] -> Mux2/1  "Zd"
  [fY] -> To Workspace2/1
  [fZ] -> To Workspace3/1
  [fPhi] -> To Workspace7/1
  [fTheta] -> To Workspace8/1
  [fPsi] -> To Workspace9/1
  [fX] -> To Workspace1/1
  Desired Values/2(Theta_d) -> To Workspace18/1, [Theta_d]
  Desired Values/4(Xd) -> [Xd], To Workspace13/1
  Desired Values/1(Phi_d) -> To Workspace17/1, [Phi_d]
  Desired Values/3(Psi_d) -> [Psi_d], To Workspace16/1
  Desired Values/6(Zd) -> [Zd], To Workspace15/1
  Clock/1 -> To Workspace/1, Desired Values/1(t)
  Desired Values/5(Yd) -> [Yd], To Workspace14/1
  Mux5/1 -> Psi_d & Psi/1
  [Psi_d] -> Mux5/1  "Psi_d"
  From37/1 -> "Theta "/1  "Theta"
  From34/1 -> " Phi "/1  "Phi"
  [fPsi] -> Mux5/2  "Psi"
  Mux7/1 -> Theta 1/1
  [Phi_d] -> Mux6/1
  [fTheta] -> Mux7/2  "Theta"
  Mux6/1 -> " Phi 1"/1
  [Theta_d] -> Mux7/1
  [fPhi] -> Mux6/2  "Phi"
  [fY] -> Mux3/2
  [fZ] -> Mux3/3
  [fX] -> Mux3/1
  Mux3/1 -> To Workspace20/1, xLeader/1
  [fX] -> Sum/2  "fx"
  [Xd] -> Sum/1  "xd"
  [fY] -> Sum1/2  "fy"
  [Yd] -> Sum1/1  "yd"
  [Zd] -> Sum2/1  "zd"
  [fZ] -> Sum2/2  "fz"
  Sum1/1 -> Mux8/2, ez/2(e_y)
  Sum/1 -> Mux8/1, ez/1(e_x)
  Sum2/1 -> ez/3(e_z), Mux8/3
  [fPhi] -> Mux4/1
  [fTheta] -> Mux4/2
  [fPsi] -> Mux4/3
  [fU1] -> Mux9/1  "fU1"
  [fU2] -> Mux9/2  "fU2"
  [fU3] -> Mux9/3  "fU3"
  [fU4] -> Mux9/4  "fU4"
  [fUx] -> Mux9/5  "fUx"
  [fUy] -> Mux9/6  "fUy"
  Mux9/1 -> To Workspace19/1
  Mux8/1 -> To Workspace21/1
  Mux4/1 -> To Workspace22/1

== system RobustFormationControl_FractionalModel_under_Dis/Fractional Leader with four followers/Follower 1 System/Desired Values ==
  t : Inport
  Helical Trajectry : Subsystem  Commented=on
  Helical Trajectry1 : Subsystem
  Step : Step  Time=0  After=0.001  SampleTime=0
  Step Inputs Trajectry : Subsystem  Commented=on
  Phi_d : Outport  VectorParamsAs1DForOutWhenUnconnected=off
  Theta_d : Outport  Port=2  VectorParamsAs1DForOutWhenUnconnected=off
  Psi_d : Outport  Port=3  VectorParamsAs1DForOutWhenUnconnected=off
  Xd : Outport  Port=4  VectorParamsAs1DForOutWhenUnconnected=off
  Yd : Outport  Port=5  VectorParamsAs1DForOutWhenUnconnected=off
  Zd : Outport  Port=6  VectorParamsAs1DForOutWhenUnconnected=off
  wires:
  t/1 -> Helical Trajectry1/1(t), Helical Trajectry/1(t)
  Step/1 -> Theta_d/1, Phi_d/1
  Helical Trajectry1/1(xd) -> Xd/1
  Helical Trajectry1/4(Psi_d) -> Psi_d/1
  Helical Trajectry1/2(yd) -> Yd/1
  Helical Trajectry1/3(zd) -> Zd/1

== system RobustFormationControl_FractionalModel_under_Dis/Fractional Leader with four followers/Follower 1 System/Follower 1 Quadrotor Model ==
  xd : Inport
  yd : Inport  Port=2
  zd : Inport  Port=3
  Psi_d : Inport  Port=4
  xLeader : Inport  Port=5
  dXYZ : Inport  Port=6
  Control Module1 : Subsystem
  Quadrotor Dynamic System : Subsystem
  X : Outport  VectorParamsAs1DForOutWhenUnconnected=off
  Y : Outport  Port=2  VectorParamsAs1DForOutWhenUnconnected=off
  Z : Outport  Port=3  VectorParamsAs1DForOutWhenUnconnected=off
  Phi : Outport  Port=4  VectorParamsAs1DForOutWhenUnconnected=off
  Theta : Outport  Port=5  VectorParamsAs1DForOutWhenUnconnected=off
  Psi : Outport  Port=6  VectorParamsAs1DForOutWhenUnconnected=off
  U1 : Outport  Port=7  VectorParamsAs1DForOutWhenUnconnected=off
  U2 : Outport  Port=8  VectorParamsAs1DForOutWhenUnconnected=off
  U3 : Outport  Port=9  VectorParamsAs1DForOutWhenUnconnected=off
  U4 : Outport  Port=10  VectorParamsAs1DForOutWhenUnconnected=off
  Ux : Outport  Port=11  VectorParamsAs1DForOutWhenUnconnected=off
  Uy : Outport  Port=12  VectorParamsAs1DForOutWhenUnconnected=off
  wires:
  Control Module1/5(Ux) -> Ux/1, Quadrotor Dynamic System/5(Ux)  "Ux"
  Quadrotor Dynamic System/2(y = x9) -> [x9], Y/1  "Y"
  Quadrotor Dynamic System/6(Psi) -> [x5], Psi/1  "Psi"
  Control Module1/4(U4) -> U4/1, Quadrotor Dynamic System/4(U4)  "U4"
  Quadrotor Dynamic System/3(z = x11) -> [x11], Z/1  "Z"
  Quadrotor Dynamic System/4(Phi) -> [x1], Phi/1  "Phi"
  Quadrotor Dynamic System/5(Theta) -> [x3], Theta/1  "Theta"
  Quadrotor Dynamic System/1(x = x7) -> [x7], X/1  "X"
  Control Module1/6(Uy) -> Uy/1, Quadrotor Dynamic System/6(Uy)  "Uy"
  Control Module1/1(U1) -> Quadrotor Dynamic System/1(U1), U1/1  "U1"
  Control Module1/2(U2) -> Quadrotor Dynamic System/2(U2), U2/1  "U2"
  Control Module1/3(U3) -> U3/1, Quadrotor Dynamic System/3(U3)  "U3"
  Control Module1/7(Omega) -> Quadrotor Dynamic System/7(Omega)
  Quadrotor Dynamic System/7(x2) -> [x2]
  Quadrotor Dynamic System/12(zdot = x12) -> [x12]
  Quadrotor Dynamic System/11(ydot = x10) -> [x10]
  Quadrotor Dynamic System/10(xdot = x8) -> [x8]
  Quadrotor Dynamic System/9(x6) -> [x6]
  Quadrotor Dynamic System/8(x4) -> [x4]
  [x1] -> Control Module1/1(x1)
  [x2] -> Control Module1/2(x2)
  [x3] -> Control Module1/3(x3)
  [x4] -> Control Module1/4(x4)
  [x5] -> Control Module1/5(x5)
  [x6] -> Control Module1/6(x6)
  [x7] -> Control Module1/7(x7)
  [x8] -> Control Module1/8(x8)
  [x9] -> Control Module1/9(x9)
  [x10] -> Control Module1/10(x10)
  [x11] -> Control Module1/11(x11)
  [x12] -> Control Module1/12(x12)
  xd/1 -> Control Module1/14(" xd")
  yd/1 -> Control Module1/15(yd)
  zd/1 -> Control Module1/16(" zd")
  Psi_d/1 -> Control Module1/13(Psi_d)
  xLeader/1 -> Control Module1/17(xLeader)
  dXYZ/1 -> Control Module1/18(Distance_d)

== system RobustFormationControl_FractionalModel_under_Dis/Fractional Leader with four followers/Follower 1 System/Results Plot ==
  note: yL
  xF : Inport
  xL : Inport  Port=2
  Demux : Demux  Outputs=3
  Demux1 : Demux  Outputs=3
  x : Scope  NumInputPorts=2
  y : Scope  NumInputPorts=2
  z : Scope  NumInputPorts=2
  wires:
  xF/1 -> Demux/1
  xL/1 -> Demux1/1
  Demux/1 -> x/1  "xF"
  Demux1/1 -> x/2  "xL"
  Demux/2 -> y/1  "yF"
  Demux1/2 -> y/2
  Demux/3 -> z/1  "zF"
  Demux1/3 -> z/2  "zL"

== system RobustFormationControl_FractionalModel_under_Dis/Fractional Leader with four followers/Follower 1 System/ez ==
  note: error analysis for x - position
  note: error analysis for z - position
  note: error analysis for y - position
  e_x : Inport
  e_y : Inport  Port=2
  e_z : Inport  Port=3
  Abs : Abs  SaturateOnIntegerOverflow=off
  Abs1 : Abs  SaturateOnIntegerOverflow=off
  Abs2 : Abs  SaturateOnIntegerOverflow=off
  Clock1 : Clock
  IAE : Display
  IAE1 : Display
  IAE2 : Display
  ISE : Display
  ISE1 : Display
  ISE2 : Display
  ITAE : Display
  ITAE1 : Display
  ITAE2 : Display
  ITSE : Display
  ITSE1 : Display
  ITSE2 : Display
  Integrator{,1..11} (12 alike) : Integrator
  Math Function : Math  Operator=square
  Math Function1 : Math  Operator=square
  Math Function2 : Math  Operator=square
  Mux : Mux
  Mux1 : Mux
  Mux2 : Mux
  Product{,1..5} (6 alike) : Product
  To Workspace : ToWorkspace  VariableName=fEx1  SampleTime=-1
  To Workspace1 : ToWorkspace  VariableName=fEz1  SampleTime=-1
  To Workspace2 : ToWorkspace  VariableName=fEy1  SampleTime=-1
  wires:
  Abs/1 -> Product/1, Integrator/1
  Integrator/1 -> Mux/1, IAE/1
  Math Function/1 -> Product1/1, Integrator1/1
  Integrator1/1 -> Mux/2, ISE/1
  Product/1 -> Integrator2/1
  Integrator2/1 -> Mux/3, ITAE/1
  Product1/1 -> Integrator3/1
  Integrator3/1 -> Mux/4, ITSE/1
  [time] -> Product1/2, Product/2
  [time] -> Product2/2, Product3/2
  Integrator7/1 -> Mux2/4, ITSE1/1
  Product3/1 -> Integrator7/1
  Integrator6/1 -> Mux2/3, ITAE1/1
  Product2/1 -> Integrator6/1
  Integrator5/1 -> Mux2/2, ISE1/1
  Math Function1/1 -> Integrator5/1, Product3/1
  Integrator4/1 -> Mux2/1, IAE1/1
  Abs1/1 -> Integrator4/1, Product2/1
  [ey] -> Abs1/1, Math Function1/1
  [ez] -> Math Function2/1, Abs2/1
  Abs2/1 -> Product4/1, Integrator8/1
  Integrator8/1 -> Mux1/1, IAE2/1
  Math Function2/1 -> Product5/1, Integrator9/1
  Integrator9/1 -> Mux1/2, ISE2/1
  Product4/1 -> Integrator10/1
  Integrator10/1 -> Mux1/3, ITAE2/1
  Product5/1 -> Integrator11/1
  Integrator11/1 -> Mux1/4, ITSE2/1
  [time] -> Product5/2, Product4/2
  e_x/1 -> [ex]
  e_y/1 -> [ey]
  e_z/1 -> [ez]
  Clock1/1 -> [time]
  [ex] -> Math Function/1, Abs/1
  Mux/1 -> To Workspace/1
  Mux1/1 -> To Workspace1/1
  Mux2/1 -> To Workspace2/1

== system RobustFormationControl_FractionalModel_under_Dis/Fractional Leader with four followers/Follower 2 System/Desired Values ==
  t : Inport
  Helical Trajectry : Subsystem  Commented=on
  Helical Trajectry1 : Subsystem
  Step : Step  Time=0  After=0.001  SampleTime=0
  Step Inputs Trajectry : Subsystem  Commented=on
  Phi_d : Outport  VectorParamsAs1DForOutWhenUnconnected=off
  Theta_d : Outport  Port=2  VectorParamsAs1DForOutWhenUnconnected=off
  Psi_d : Outport  Port=3  VectorParamsAs1DForOutWhenUnconnected=off
  Xd : Outport  Port=4  VectorParamsAs1DForOutWhenUnconnected=off
  Yd : Outport  Port=5  VectorParamsAs1DForOutWhenUnconnected=off
  Zd : Outport  Port=6  VectorParamsAs1DForOutWhenUnconnected=off
  wires:
  t/1 -> Helical Trajectry1/1(t), Helical Trajectry/1(t)
  Step/1 -> Theta_d/1, Phi_d/1
  Helical Trajectry1/1(xd) -> Xd/1
  Helical Trajectry1/4(Psi_d) -> Psi_d/1
  Helical Trajectry1/2(yd) -> Yd/1
  Helical Trajectry1/3(zd) -> Zd/1

== system RobustFormationControl_FractionalModel_under_Dis/Fractional Leader with four followers/Follower 2 System/Follower 2 Quadrotor Model ==
  xd : Inport
  yd : Inport  Port=2
  zd : Inport  Port=3
  Psi_d : Inport  Port=4
  xLeader : Inport  Port=5
  dXYZ : Inport  Port=6
  Control Module1 : Subsystem
  Quadrotor Dynamic System : Subsystem
  X : Outport  VectorParamsAs1DForOutWhenUnconnected=off
  Y : Outport  Port=2  VectorParamsAs1DForOutWhenUnconnected=off
  Z : Outport  Port=3  VectorParamsAs1DForOutWhenUnconnected=off
  Phi : Outport  Port=4  VectorParamsAs1DForOutWhenUnconnected=off
  Theta : Outport  Port=5  VectorParamsAs1DForOutWhenUnconnected=off
  Psi : Outport  Port=6  VectorParamsAs1DForOutWhenUnconnected=off
  U1 : Outport  Port=7  VectorParamsAs1DForOutWhenUnconnected=off
  U2 : Outport  Port=8  VectorParamsAs1DForOutWhenUnconnected=off
  U3 : Outport  Port=9  VectorParamsAs1DForOutWhenUnconnected=off
  U4 : Outport  Port=10  VectorParamsAs1DForOutWhenUnconnected=off
  Ux : Outport  Port=11  VectorParamsAs1DForOutWhenUnconnected=off
  Uy : Outport  Port=12  VectorParamsAs1DForOutWhenUnconnected=off
  wires:
  Control Module1/5(Ux) -> Ux/1, Quadrotor Dynamic System/5(Ux)  "Ux"
  Quadrotor Dynamic System/2(y = x9) -> [x9], Y/1  "Y"
  Quadrotor Dynamic System/6(Psi) -> [x5], Psi/1  "Psi"
  Control Module1/4(U4) -> U4/1, Quadrotor Dynamic System/4(U4)  "U4"
  Quadrotor Dynamic System/3(z = x11) -> [x11], Z/1  "Z"
  Quadrotor Dynamic System/4(Phi) -> [x1], Phi/1  "Phi"
  Quadrotor Dynamic System/5(Theta) -> [x3], Theta/1  "Theta"
  Quadrotor Dynamic System/1(x = x7) -> [x7], X/1  "X"
  Control Module1/6(Uy) -> Uy/1, Quadrotor Dynamic System/6(Uy)  "Uy"
  Control Module1/1(U1) -> Quadrotor Dynamic System/1(U1), U1/1  "U1"
  Control Module1/2(U2) -> U2/1, Quadrotor Dynamic System/2(U2)  "U2"
  Control Module1/3(U3) -> U3/1, Quadrotor Dynamic System/3(U3)  "U3"
  Control Module1/7(Omega) -> Quadrotor Dynamic System/7(Omega)
  Quadrotor Dynamic System/7(x2) -> [x2]
  Quadrotor Dynamic System/12(zdot = x12) -> [x12]
  Quadrotor Dynamic System/11(ydot = x10) -> [x10]
  Quadrotor Dynamic System/10(xdot = x8) -> [x8]
  Quadrotor Dynamic System/9(x6) -> [x6]
  Quadrotor Dynamic System/8(x4) -> [x4]
  [x1] -> Control Module1/1(x1)
  [x2] -> Control Module1/2(x2)
  [x3] -> Control Module1/3(x3)
  [x4] -> Control Module1/4(x4)
  [x5] -> Control Module1/5(x5)
  [x6] -> Control Module1/6(x6)
  [x7] -> Control Module1/7(x7)
  [x8] -> Control Module1/8(x8)
  [x9] -> Control Module1/9(x9)
  [x10] -> Control Module1/10(x10)
  [x11] -> Control Module1/11(x11)
  [x12] -> Control Module1/12(x12)
  xd/1 -> Control Module1/14(" xd")
  yd/1 -> Control Module1/15(yd)
  zd/1 -> Control Module1/16(" zd")
  Psi_d/1 -> Control Module1/13(Psi_d)
  xLeader/1 -> Control Module1/17(xLeader)
  dXYZ/1 -> Control Module1/18(Distance_d)

== system RobustFormationControl_FractionalModel_under_Dis/Fractional Leader with four followers/Follower 2 System/Results Plot ==
  note: yL
  xF : Inport
  xL : Inport  Port=2
  Demux : Demux  Outputs=3
  Demux1 : Demux  Outputs=3
  x : Scope  NumInputPorts=2
  y : Scope  NumInputPorts=2
  z : Scope  NumInputPorts=2
  wires:
  xF/1 -> Demux/1
  xL/1 -> Demux1/1
  Demux/1 -> x/1  "xF"
  Demux1/1 -> x/2  "xL"
  Demux/2 -> y/1  "yF"
  Demux1/2 -> y/2
  Demux/3 -> z/1  "zF"
  Demux1/3 -> z/2  "zL"

== system RobustFormationControl_FractionalModel_under_Dis/Fractional Leader with four followers/Follower 2 System/ez ==
  note: error analysis for x - position
  note: error analysis for z - position
  note: error analysis for y - position
  e_x : Inport
  e_y : Inport  Port=2
  e_z : Inport  Port=3
  Abs : Abs  SaturateOnIntegerOverflow=off
  Abs1 : Abs  SaturateOnIntegerOverflow=off
  Abs2 : Abs  SaturateOnIntegerOverflow=off
  Clock1 : Clock
  IAE : Display
  IAE1 : Display
  IAE2 : Display
  ISE : Display
  ISE1 : Display
  ISE2 : Display
  ITAE : Display
  ITAE1 : Display
  ITAE2 : Display
  ITSE : Display
  ITSE1 : Display
  ITSE2 : Display
  Integrator{,1..11} (12 alike) : Integrator
  Math Function : Math  Operator=square
  Math Function1 : Math  Operator=square
  Math Function2 : Math  Operator=square
  Mux : Mux
  Mux1 : Mux
  Mux2 : Mux
  Product{,1..5} (6 alike) : Product
  To Workspace : ToWorkspace  VariableName=fEx2  SampleTime=-1
  To Workspace1 : ToWorkspace  VariableName=fEz2  SampleTime=-1
  To Workspace2 : ToWorkspace  VariableName=fEy2  SampleTime=-1
  wires:
  Abs/1 -> Product/1, Integrator/1
  Integrator/1 -> Mux/1, IAE/1
  Math Function/1 -> Product1/1, Integrator1/1
  Integrator1/1 -> Mux/2, ISE/1
  Product/1 -> Integrator2/1
  Integrator2/1 -> Mux/3, ITAE/1
  Product1/1 -> Integrator3/1
  Integrator3/1 -> Mux/4, ITSE/1
  [time] -> Product1/2, Product/2
  [time] -> Product2/2, Product3/2
  Integrator7/1 -> Mux2/4, ITSE1/1
  Product3/1 -> Integrator7/1
  Integrator6/1 -> Mux2/3, ITAE1/1
  Product2/1 -> Integrator6/1
  Integrator5/1 -> Mux2/2, ISE1/1
  Math Function1/1 -> Integrator5/1, Product3/1
  Integrator4/1 -> Mux2/1, IAE1/1
  Abs1/1 -> Integrator4/1, Product2/1
  [ey] -> Abs1/1, Math Function1/1
  [ez] -> Math Function2/1, Abs2/1
  Abs2/1 -> Product4/1, Integrator8/1
  Integrator8/1 -> Mux1/1, IAE2/1
  Math Function2/1 -> Product5/1, Integrator9/1
  Integrator9/1 -> Mux1/2, ISE2/1
  Product4/1 -> Integrator10/1
  Integrator10/1 -> Mux1/3, ITAE2/1
  Product5/1 -> Integrator11/1
  Integrator11/1 -> Mux1/4, ITSE2/1
  [time] -> Product5/2, Product4/2
  e_x/1 -> [ex]
  e_y/1 -> [ey]
  e_z/1 -> [ez]
  Clock1/1 -> [time]
  [ex] -> Math Function/1, Abs/1
  Mux/1 -> To Workspace/1
  Mux1/1 -> To Workspace1/1
  Mux2/1 -> To Workspace2/1

== system RobustFormationControl_FractionalModel_under_Dis/Fractional Leader with four followers/Follower 3 System/Desired Values ==
  t : Inport
  Helical Trajectry : Subsystem  Commented=on
  Helical Trajectry1 : Subsystem
  Step : Step  Time=0  After=0.001  SampleTime=0
  Step Inputs Trajectry : Subsystem  Commented=on
  Phi_d : Outport  VectorParamsAs1DForOutWhenUnconnected=off
  Theta_d : Outport  Port=2  VectorParamsAs1DForOutWhenUnconnected=off
  Psi_d : Outport  Port=3  VectorParamsAs1DForOutWhenUnconnected=off
  Xd : Outport  Port=4  VectorParamsAs1DForOutWhenUnconnected=off
  Yd : Outport  Port=5  VectorParamsAs1DForOutWhenUnconnected=off
  Zd : Outport  Port=6  VectorParamsAs1DForOutWhenUnconnected=off
  wires:
  Helical Trajectry1/3(zd) -> Zd/1
  Helical Trajectry1/2(yd) -> Yd/1
  Helical Trajectry1/4(Psi_d) -> Psi_d/1
  Helical Trajectry1/1(xd) -> Xd/1
  Step/1 -> Phi_d/1, Theta_d/1
  t/1 -> Helical Trajectry1/1(t), Helical Trajectry/1(t)
